simulink model "Switch_PWM"  (R2022a)
settings: Solver=FixedStepAuto  StartTime=0.0  StopTime=0.1  FixedStep=1e-7  RelTol=1e-3
libraries: simulink x2, spspowerguiLib x1
settings Model: Creator=Bobby  LastModifiedBy=Bobby

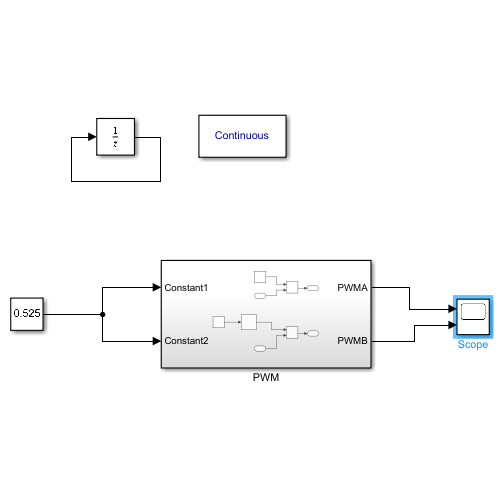
[thumbnail: Simulink's stored preview of the top-level diagram]
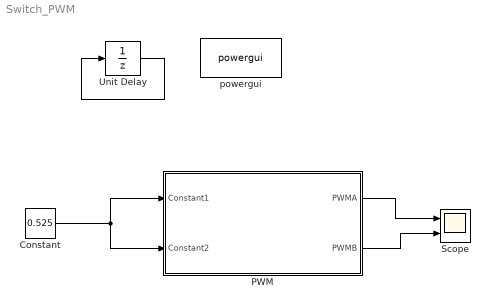
== system Switch_PWM ==
  Constant : Constant  Value=0.525
  PWM : Subsystem
  Scope : Scope  NumInputPorts=2
  Unit Delay : UnitDelay  SampleTime=-1  HasFrameUpgradeWarning=on
  powergui : spspowerguiLib/powergui  Priority=1  SimulationMode=Continuous  SampleTime=50e-6  frequency=60  Iterations=50  frequencyindice=60  Pbase=100e6  ErrMax=1e-4  UnitsV=kV  UnitsW=MW  buscounter=0  FunctionMessages=off  echomessages=off  EnableUseOfTLC=off  CurrentSourceSwitches=off  DisableSnubberDevices=off  DisableRonSwitches=off  DisableVfSwitches=off  DisplayEquations=off  AutomaticDiscreteSolvers=off  SolverType=Tustin/Backward Euler (TBE)  Interpol=off  ExternalGateDelay=off  methode=off  Ts=100  x0status=blocks  SPID=on  SwTol=0  HookPort=off  NonlinearTolerance=1e-4  nMaxIteration=100  ContinueOnMaxIteration=off  RestoreLinks=warning  ResistiveCurrentMeasurement=off  Frange=[0:2:500]  Ylog=off  Xlog=on  ShowGrid=off  save=off  variable=ZData  structure=0  ZoomFFT=off  StartTime=0.0  cycles=1  DisplayStyle=1  fundamental=60  FreqAxis=off  MaxFrequency=1000  frequencyindicesteady=1  RmsSteady=1  display=off
  wires:
  Unit Delay/1 -> Unit Delay/1
  Constant/1 -> PWM/2(Constant2), PWM/1(Constant1)
  PWM/1(PWMA) -> Scope/1
  PWM/2(PWMB) -> Scope/2

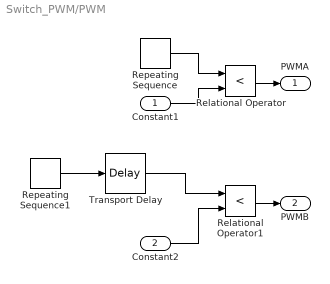
== system Switch_PWM/PWM ==
  Constant1 : Inport
  Constant2 : Inport  Port=2
  Relational Operator : RelationalOperator  Operator=<  OutDataTypeStr=boolean  RndMeth=Simplest  InputSameDT=off
  Relational Operator1 : RelationalOperator  Operator=<  OutDataTypeStr=boolean  RndMeth=Simplest  InputSameDT=off
  Repeating Sequence : simulink/Sources/Repeating Sequence  rep_seq_t=[0, 1e-5,2e-5]  rep_seq_y=[0,1,0]
  Repeating Sequence1 : simulink/Sources/Repeating Sequence  rep_seq_t=[0, 1e-5,2e-5]  rep_seq_y=[0,1,0]
  Transport Delay : TransportDelay  DelayTime=1e-5
  PWMA : Outport
  PWMB : Outport  Port=2
  wires:
  Repeating Sequence/1 -> Relational Operator/1
  Constant1/1 -> Relational Operator/2
  Constant2/1 -> Relational Operator1/2
  Transport Delay/1 -> Relational Operator1/1
  Repeating Sequence1/1 -> Transport Delay/1
  Relational Operator1/1 -> PWMB/1
  Relational Operator/1 -> PWMA/1
